simulink model "ntc_measure"  (R2024a)
settings: Solver=ode1be  StartTime=0.0  StopTime=simlength  FixedStep=tc  RelTol=1e-3
undefined symbols (not defined in the file or in its folder): open_loop_gain_opa350, Rntc, tc
libraries: fl_lib x177, ee_lib x28, nesl_utility x26
(part 1 of 2)
settings Model: SimulationMode=accelerator  Creator=ltnbda  LastModifiedBy=ltnbda
settings DataIOCC: SaveOutput=off  SignalLogging=off  DSMLogging=off  SaveTime=off  ReturnWorkspaceOutputs=off
settings RTWCC: GPUComputeCapability=3.5

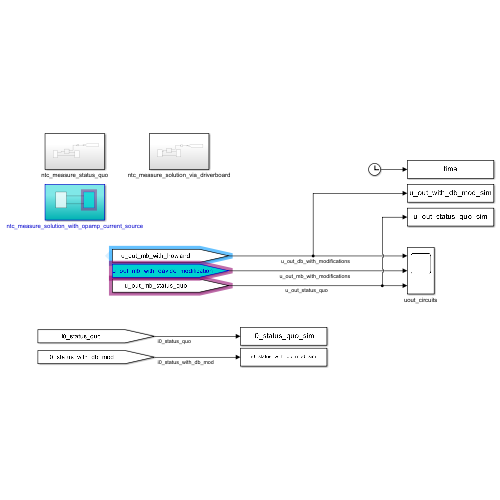
[thumbnail: Simulink's stored preview of the top-level diagram]
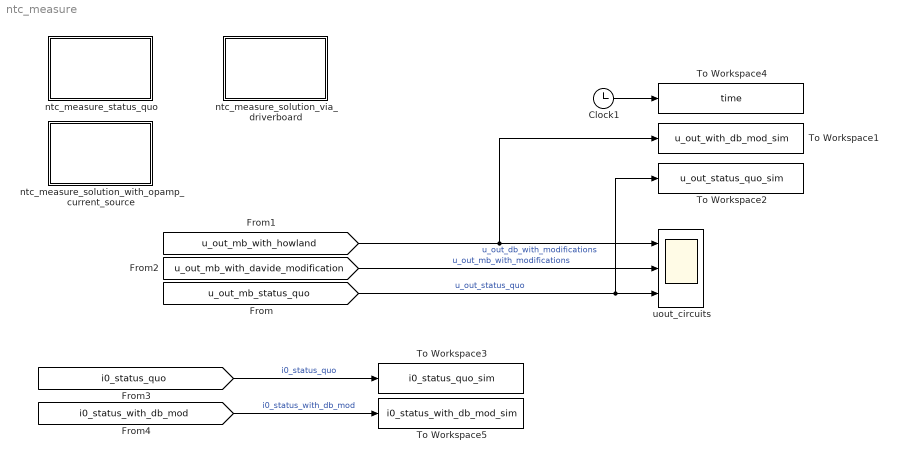
== system ntc_measure ==
  Clock1 : Clock
  To Workspace1 : ToWorkspace  VariableName=u_out_with_db_mod_sim  SampleTime=tc
      settings: MaxDataPoints=Nc
  To Workspace2 : ToWorkspace  VariableName=u_out_status_quo_sim  SampleTime=tc
      settings: MaxDataPoints=Nc
  To Workspace3 : ToWorkspace  VariableName=i0_status_quo_sim  SampleTime=tc
      settings: MaxDataPoints=Nc
  To Workspace4 : ToWorkspace  VariableName=time  SampleTime=tc
      settings: MaxDataPoints=Nc
  To Workspace5 : ToWorkspace  VariableName=i0_status_with_db_mod_sim  SampleTime=tc
      settings: MaxDataPoints=Nc
  ntc_measure_solution_via_driverboard : Subsystem
  ntc_measure_solution_with_opamp_current_source : Subsystem
  ntc_measure_status_quo : Subsystem
  uout_circuits : Scope  NumInputPorts=3
  wires:
  [u_out_mb_with_howland] -> To Workspace1/1, uout_circuits/1  "u_out_db_with_modifications"
  [u_out_mb_with_davide_modification] -> uout_circuits/2  "u_out_mb_with_modifications"
  [u_out_mb_status_quo] -> To Workspace2/1, uout_circuits/3  "u_out_status_quo"
  Clock1/1 -> To Workspace4/1
  [i0_status_quo] -> To Workspace3/1  "i0_status_quo"
  [i0_status_with_db_mod] -> To Workspace5/1  "i0_status_with_db_mod"

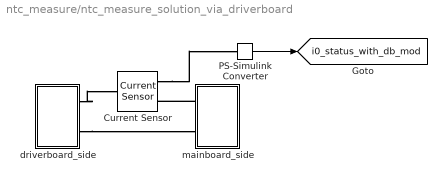
== system ntc_measure/ntc_measure_solution_via_driverboard ==
  Current Sensor : fl_lib/Electrical/Electrical Sensors/Current Sensor
  PS-Simulink Converter : nesl_utility/PS-Simulink Converter  PhysicalDomain=network_engine_domain  SubClassName=ps_output  LeftPortType=input  RightPortType=output  PseudoPeriodic=off  Frequencies=[]  VectorFormat=1-D array  Unit=A  AffineConversion=off
  driverboard_side : Subsystem
  mainboard_side : Subsystem
  tag scope: i0_status_with_db_mod=global
  wires:
  PS-Simulink Converter/1 -> [i0_status_with_db_mod]
  connections:
  driverboard_side/RConn2 -- mainboard_side/LConn2
  Current Sensor/RConn1 -- PS-Simulink Converter/LConn1
  mainboard_side/LConn1 -- Current Sensor/RConn2
  driverboard_side/RConn1 -- Current Sensor/LConn1

== system ntc_measure/ntc_measure_solution_with_opamp_current_source ==
  driverboard_side : Subsystem
  mainboard_side : Subsystem
  connections:
  mainboard_side/LConn2 -- driverboard_side/RConn2
  mainboard_side/LConn1 -- driverboard_side/RConn1

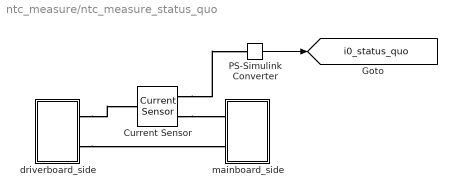
== system ntc_measure/ntc_measure_status_quo ==
  Current Sensor : fl_lib/Electrical/Electrical Sensors/Current Sensor
  PS-Simulink Converter : nesl_utility/PS-Simulink Converter  PhysicalDomain=network_engine_domain  SubClassName=ps_output  LeftPortType=input  RightPortType=output  PseudoPeriodic=off  Frequencies=[]  VectorFormat=1-D array  Unit=A  AffineConversion=off
  driverboard_side : Subsystem
  mainboard_side : Subsystem
  tag scope: i0_status_quo=global
  wires:
  PS-Simulink Converter/1 -> [i0_status_quo]
  connections:
  driverboard_side/RConn2 -- mainboard_side/LConn2
  driverboard_side/RConn1 -- Current Sensor/LConn1
  Current Sensor/RConn2 -- mainboard_side/LConn1
  Current Sensor/RConn1 -- PS-Simulink Converter/LConn1

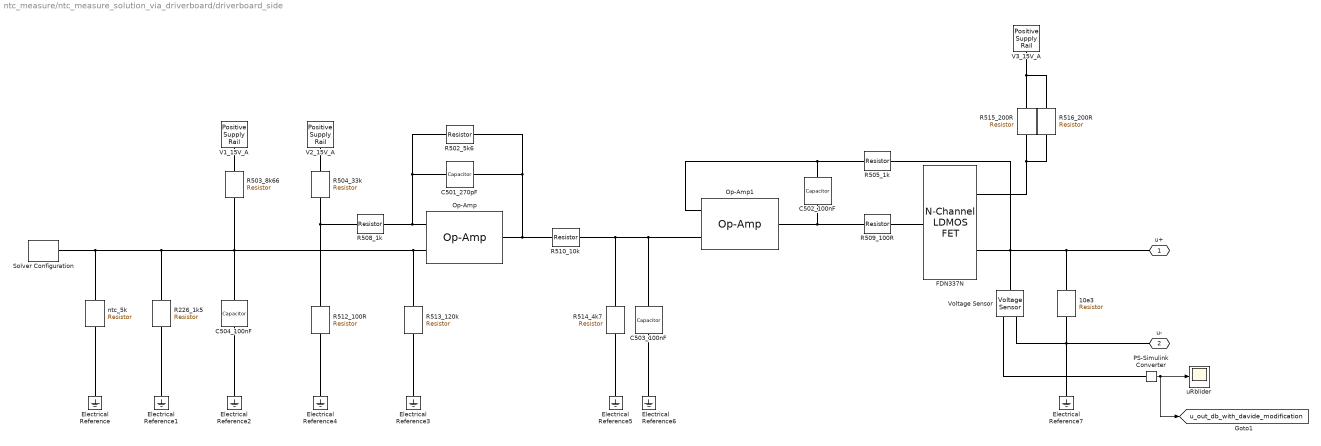
== system ntc_measure/ntc_measure_solution_via_driverboard/driverboard_side ==
  10e3 : fl_lib/Electrical/Electrical Elements/Resistor  R=10e3 Ohm  i_specify=off  i_priority=None  i=0 A  i_nominal_specify=off  i_nominal_value=1  i_nominal_unit=A  v_specify=off  v_priority=None  v=0 V  v_nominal_specify=off  v_nominal_value=1  v_nominal_unit=V
  C501_270pF : fl_lib/Electrical/Electrical Elements/Capacitor  c=270e-12 F  r=1e-6 Ohm  g=0 1/Ohm  i_specify=off  i_priority=None  i=0 A  i_nominal_specify=off  i_nominal_value=1  i_nominal_unit=A  v_specify=off  v_priority=None  v=0 V  v_nominal_specify=off  v_nominal_value=1  v_nominal_unit=V  vc_specify=off  vc_priority=High  vc=0 V  vc_nominal_specify=off  vc_nominal_value=1  vc_nominal_unit=V
  C502_100nF : fl_lib/Electrical/Electrical Elements/Capacitor  c=100e-9 F  r=1e-6 Ohm  g=0 1/Ohm  i_specify=off  i_priority=None  i=0 A  i_nominal_specify=off  i_nominal_value=1  i_nominal_unit=A  v_specify=off  v_priority=None  v=0 V  v_nominal_specify=off  v_nominal_value=1  v_nominal_unit=V  vc_specify=off  vc_priority=High  vc=0 V  vc_nominal_specify=off  vc_nominal_value=1  vc_nominal_unit=V
  C503_100nF : fl_lib/Electrical/Electrical Elements/Capacitor  c=100e-9 F  r=1e-6 Ohm  g=0 1/Ohm  i_specify=off  i_priority=None  i=0 A  i_nominal_specify=off  i_nominal_value=1  i_nominal_unit=A  v_specify=off  v_priority=None  v=0 V  v_nominal_specify=off  v_nominal_value=1  v_nominal_unit=V  vc_specify=off  vc_priority=High  vc=0 V  vc_nominal_specify=off  vc_nominal_value=1  vc_nominal_unit=V
  C504_100nF : fl_lib/Electrical/Electrical Elements/Capacitor  c=100e-9 F  r=1e-6 Ohm  g=0 1/Ohm  i_specify=off  i_priority=None  i=0 A  i_nominal_specify=off  i_nominal_value=1  i_nominal_unit=A  v_specify=off  v_priority=None  v=0 V  v_nominal_specify=off  v_nominal_value=1  v_nominal_unit=V  vc_specify=off  vc_priority=High  vc=0 V  vc_nominal_specify=off  vc_nominal_value=1  vc_nominal_unit=V
  Electrical Reference{,1..7} (8 alike) : fl_lib/Electrical/Electrical Elements/Electrical Reference
  FDN337N : ee_lib/Semiconductors & Converters/N-Channel LDMOS FET  betaref=[11.6, .01] A/V^2  Vfbref=[-1.05, -.1] V  gamma=[3.4, 2.5] V^(1/2)  phib2ref=[.95, .95] V  thesatref=[0, .1] 1/V  theaccdr=0 1/V  alpha=0  Vp=5e-2 V  m=8  Tmeas=25 degC  Rsref=1e-4 Ohm  Rdref=0.07 Ohm  Rgref=8.4 Ohm  Rdriftref=0.1 Ohm  lambda=0.2  Cox=[1600, 1000] pF  Cgso=15 pF  Cgdo=15 pF  Isref=1e-13 A  Vbi=0.6 V  n=1  Cj0=1800 pF  TT=50e-9 s  Tprm=1  Tsim=25 degC  etabet=[1.3, 1.3]  Stvfb=[.0005, .0005] V/K  Stphib=-8.5e-4 V/K  etasat=[1.04, 1.04]  etar=0.95  etardr=0.95  etais=3  Ig_specify=off  Ig_priority=None  Ig=0 A  Ig_nominal_specify=off  Ig_nominal_value=1  Ig_nominal_unit=A  Id_specify=off  Id_priority=None  Id=0 A  Id_nominal_specify=off  Id_nominal_value=1  Id_nominal_unit=A  V_gs_specify=off  V_gs_priority=None  V_gs=0 V  V_gs_nominal_specify=off  V_gs_nominal_value=1  V_gs_nominal_unit=V  V_ds_specify=off  V_ds_priority=None  V_ds=0 V  V_ds_nominal_specify=off  V_ds_nominal_value=1  V_ds_nominal_unit=V  QGoverCox_specify=off  QGoverCox_priority=Low  QGoverCox=0 V  QGoverCox_nominal_specify=off  QGoverCox_nominal_value=1  QGoverCox_nominal_unit=V  QDoverCox_specify=off  QDoverCox_priority=Low  QDoverCox=0 V  QDoverCox_nominal_specify=off  QDoverCox_nominal_value=1  QDoverCox_nominal_unit=V  thermal_network_parameterization=ee.enum.thermalNetworkTopology.junctionCase  Rth=[0, 10] K/W  Rth_Cauer=[1, 3, 10] K/W  Rth_Foster=[4, 6] K/W  thermal_mass_parameterization=ee.enum.thermalNetwork.timeconstant  thermal_mass=[0, 1] J/K  thermal_mass_Cauer=[.1, .3, 1] J/K  thermal_mass_Foster=[1.5, 3] J/K  thermal_time_constant=[0, 10] s  thermal_time_constant_Cauer=[1, 3, 10] s  thermal_time_constant_Foster=[6, 18] s  T0=[25, 25] degC  T0_Cauer=[25, 25, 25] degC  Tvec_initial_Foster=[25, 25, 25, 25] degC
      settings: InternalSimscapePortConfiguration="{\"Bottom\":[],\"Left\":[{\"id\":\"G\",\"label\":\"\",\"type\":\"foundation.electrical.electrical\"}],\"Right\":[{\"id\":\"D\",\"label\":\"d\",\"type\":\"foundation.electrical.electrical\"},{\"id\":\"S\",\"label\":\"s\",\"type\":\"foundation.electrical.electrical\"}],\"Top\":[]}"
  Op-Amp : fl_lib/Electrical/Electrical Elements/Op-Amp  outI_specify=off  outI_priority=None  outI=0 A  outI_nominal_specify=off  outI_nominal_value=1  outI_nominal_unit=A
  Op-Amp1 : fl_lib/Electrical/Electrical Elements/Op-Amp  outI_specify=off  outI_priority=None  outI=0 A  outI_nominal_specify=off  outI_nominal_value=1  outI_nominal_unit=A
  PS-Simulink Converter : nesl_utility/PS-Simulink Converter  PhysicalDomain=network_engine_domain  SubClassName=ps_output  LeftPortType=input  RightPortType=output  PseudoPeriodic=off  Frequencies=[]  VectorFormat=1-D array  Unit=V  AffineConversion=off
  R226_1k5 : fl_lib/Electrical/Electrical Elements/Resistor  R=1.5e3 Ohm  i_specify=off  i_priority=None  i=0 A  i_nominal_specify=off  i_nominal_value=1  i_nominal_unit=A  v_specify=off  v_priority=None  v=0 V  v_nominal_specify=off  v_nominal_value=1  v_nominal_unit=V
  R502_5k6 : fl_lib/Electrical/Electrical Elements/Resistor  R=5.6e3 Ohm  i_specify=off  i_priority=None  i=0 A  i_nominal_specify=off  i_nominal_value=1  i_nominal_unit=A  v_specify=off  v_priority=None  v=0 V  v_nominal_specify=off  v_nominal_value=1  v_nominal_unit=V
  R503_8k66 : fl_lib/Electrical/Electrical Elements/Resistor  R=8.66e3 Ohm  i_specify=off  i_priority=None  i=0 A  i_nominal_specify=off  i_nominal_value=1  i_nominal_unit=A  v_specify=off  v_priority=None  v=0 V  v_nominal_specify=off  v_nominal_value=1  v_nominal_unit=V
  R504_33k : fl_lib/Electrical/Electrical Elements/Resistor  R=33e3 Ohm  i_specify=off  i_priority=None  i=0 A  i_nominal_specify=off  i_nominal_value=1  i_nominal_unit=A  v_specify=off  v_priority=None  v=0 V  v_nominal_specify=off  v_nominal_value=1  v_nominal_unit=V
  R505_1k : fl_lib/Electrical/Electrical Elements/Resistor  R=1e3 Ohm  i_specify=off  i_priority=None  i=0 A  i_nominal_specify=off  i_nominal_value=1  i_nominal_unit=A  v_specify=off  v_priority=None  v=0 V  v_nominal_specify=off  v_nominal_value=1  v_nominal_unit=V
  R508_1k : fl_lib/Electrical/Electrical Elements/Resistor  R=1e3 Ohm  i_specify=off  i_priority=None  i=0 A  i_nominal_specify=off  i_nominal_value=1  i_nominal_unit=A  v_specify=off  v_priority=None  v=0 V  v_nominal_specify=off  v_nominal_value=1  v_nominal_unit=V
  R509_100R : fl_lib/Electrical/Electrical Elements/Resistor  R=100 Ohm  i_specify=off  i_priority=None  i=0 A  i_nominal_specify=off  i_nominal_value=1  i_nominal_unit=A  v_specify=off  v_priority=None  v=0 V  v_nominal_specify=off  v_nominal_value=1  v_nominal_unit=V
  R510_10k : fl_lib/Electrical/Electrical Elements/Resistor  R=10e3 Ohm  i_specify=off  i_priority=None  i=0 A  i_nominal_specify=off  i_nominal_value=1  i_nominal_unit=A  v_specify=off  v_priority=None  v=0 V  v_nominal_specify=off  v_nominal_value=1  v_nominal_unit=V
  R512_100R : fl_lib/Electrical/Electrical Elements/Resistor  R=100 Ohm  i_specify=off  i_priority=None  i=0 A  i_nominal_specify=off  i_nominal_value=1  i_nominal_unit=A  v_specify=off  v_priority=None  v=0 V  v_nominal_specify=off  v_nominal_value=1  v_nominal_unit=V
  R513_120k : fl_lib/Electrical/Electrical Elements/Resistor  R=120e3 Ohm  i_specify=off  i_priority=None  i=0 A  i_nominal_specify=off  i_nominal_value=1  i_nominal_unit=A  v_specify=off  v_priority=None  v=0 V  v_nominal_specify=off  v_nominal_value=1  v_nominal_unit=V
  R514_4k7 : fl_lib/Electrical/Electrical Elements/Resistor  R=4.7e3 Ohm  i_specify=off  i_priority=None  i=0 A  i_nominal_specify=off  i_nominal_value=1  i_nominal_unit=A  v_specify=off  v_priority=None  v=0 V  v_nominal_specify=off  v_nominal_value=1  v_nominal_unit=V
  R515_200R : fl_lib/Electrical/Electrical Elements/Resistor  R=200 Ohm  i_specify=off  i_priority=None  i=0 A  i_nominal_specify=off  i_nominal_value=1  i_nominal_unit=A  v_specify=off  v_priority=None  v=0 V  v_nominal_specify=off  v_nominal_value=1  v_nominal_unit=V
  R516_200R : fl_lib/Electrical/Electrical Elements/Resistor  R=200 Ohm  i_specify=off  i_priority=None  i=0 A  i_nominal_specify=off  i_nominal_value=1  i_nominal_unit=A  v_specify=off  v_priority=None  v=0 V  v_nominal_specify=off  v_nominal_value=1  v_nominal_unit=V
  Solver Configuration : nesl_utility/Solver Configuration  PhysicalDomain=network_engine_domain  SubClassName=solver  LeftPortType=input  RightPortType=generic  Tones=[]  Harmonics=[]  SimulateNoise=off  Profile=off  UseLocalSampling=off  EnableSwitchedLinearOptims=on  FrequencyDomain=off  UseCCode=off  RelTol=0.001  AbsTol=0.001  MinStep=1e-09  ToWorkspace=off  RevertToSquareIcSolve=off  NumHomotopyIterations=100  PhasorMode=off  PhasorModeNumHarmonics=1  ConsistencySolver=NEWTON_XTOL_AFTER_FTOL  IndexReductionMethod=DerivativeReplacement  DoDC=off  ResidualTolerance=1e-09  ConsistencyTolSource=GLOBAL  ConsistencyAbsTol=0.001  ConsistencyRelTol=0.001  ConsistencyTolFactor=0.001  UseLocalSolver=on  LocalSolverChoice=NE_BACKWARD_EULER_ADVANCER  ResolveIndetEquations=on  FunctionEvalNumThread=1  LocalSolverSampleTime=tc  DoFixedCost=on  MaxNonlinIter=3  MaxModeIter=2  ComputeImpulses=off  ImpulseIterations=2  LinearAlgebra=auto  LinearAlgebraNumThread=0  EquationFormulation=NE_TIME_EF  DelaysMemoryBudget=1024  AutomaticFiltering=on  FilteringTimeConstant=0.001  PartitionStorageMethod=AS_NEEDED  PartitionMemoryBudget=1024  PartitionMethod=ROBUST  MultibodyUseLocalSolver=off  MultibodyLocalSolverChoice=ODE1  MultibodyLocalSolverSampleTime=0.001
  V1_15V_A : ee_lib/Sources/Positive Supply Rail  v0=15 V
      settings: InternalSimscapePortConfiguration="{\"Bottom\":[],\"Left\":[],\"Right\":[{\"id\":\"p\",\"label\":\"\",\"type\":\"foundation.electrical.electrical\"}],\"Top\":[]}"
  V2_15V_A : ee_lib/Sources/Positive Supply Rail  v0=15 V
      settings: InternalSimscapePortConfiguration="{\"Bottom\":[],\"Left\":[],\"Right\":[{\"id\":\"p\",\"label\":\"\",\"type\":\"foundation.electrical.electrical\"}],\"Top\":[]}"
  V3_15V_A : ee_lib/Sources/Positive Supply Rail  v0=15 V
      settings: InternalSimscapePortConfiguration="{\"Bottom\":[],\"Left\":[],\"Right\":[{\"id\":\"p\",\"label\":\"\",\"type\":\"foundation.electrical.electrical\"}],\"Top\":[]}"
  Voltage Sensor : fl_lib/Electrical/Electrical Sensors/Voltage Sensor
  ntc_5k : fl_lib/Electrical/Electrical Elements/Resistor  R=Rntc Ohm  i_specify=off  i_priority=None  i=0 A  i_nominal_specify=off  i_nominal_value=1  i_nominal_unit=A  v_specify=off  v_priority=None  v=0 V  v_nominal_specify=off  v_nominal_value=1  v_nominal_unit=V
  uRblider : Scope
  u+ : PMIOPort  Side=Right
  u- : PMIOPort  Port=2  Side=Right
  tag scope: u_out_db_with_davide_modification=global
  wires:
  PS-Simulink Converter/1 -> [u_out_db_with_davide_modification], uRblider/1
  connections:
  PS-Simulink Converter/LConn1 -- Voltage Sensor/RConn1
  Electrical Reference4/LConn1 -- R512_100R/RConn1
  Electrical Reference3/LConn1 -- R513_120k/RConn1
  Electrical Reference6/LConn1 -- C503_100nF/RConn1
  R502_5k6/RConn1 -- Op-Amp/RConn1 -- R510_10k/LConn1 -- C501_270pF/RConn1
  R514_4k7/LConn1 -- Op-Amp1/LConn1 -- C503_100nF/LConn1 -- R510_10k/RConn1
  Electrical Reference2/LConn1 -- C504_100nF/RConn1
  Electrical Reference1/LConn1 -- R226_1k5/RConn1
  V1_15V_A/RConn1 -- R503_8k66/LConn1
  Electrical Reference/LConn1 -- ntc_5k/RConn1
  R509_100R/LConn1 -- C502_100nF/RConn1 -- Op-Amp1/RConn1
  u+/RConn1 -- 10e3/LConn1 -- FDN337N/RConn2 -- Voltage Sensor/LConn1 -- R505_1k/RConn1
  FDN337N/LConn1 -- R509_100R/RConn1
  C501_270pF/LConn1 -- R502_5k6/LConn1 -- Op-Amp/LConn2 -- R508_1k/RConn1
  R505_1k/LConn1 -- C502_100nF/LConn1 -- Op-Amp1/LConn2
  R504_33k/LConn1 -- V2_15V_A/RConn1
  Voltage Sensor/RConn2 -- Electrical Reference7/LConn1 -- 10e3/RConn1 -- u-/RConn1
  Electrical Reference5/LConn1 -- R514_4k7/RConn1
  C504_100nF/LConn1 -- R513_120k/LConn1 -- Op-Amp/LConn1 -- Solver Configuration/RConn1 -- ntc_5k/LConn1 -- R226_1k5/LConn1 -- R503_8k66/RConn1
  R504_33k/RConn1 -- R512_100R/LConn1 -- R508_1k/LConn1
  R515_200R/LConn1 -- R516_200R/LConn1 -- V3_15V_A/RConn1
  FDN337N/RConn1 -- R516_200R/RConn1 -- R515_200R/RConn1

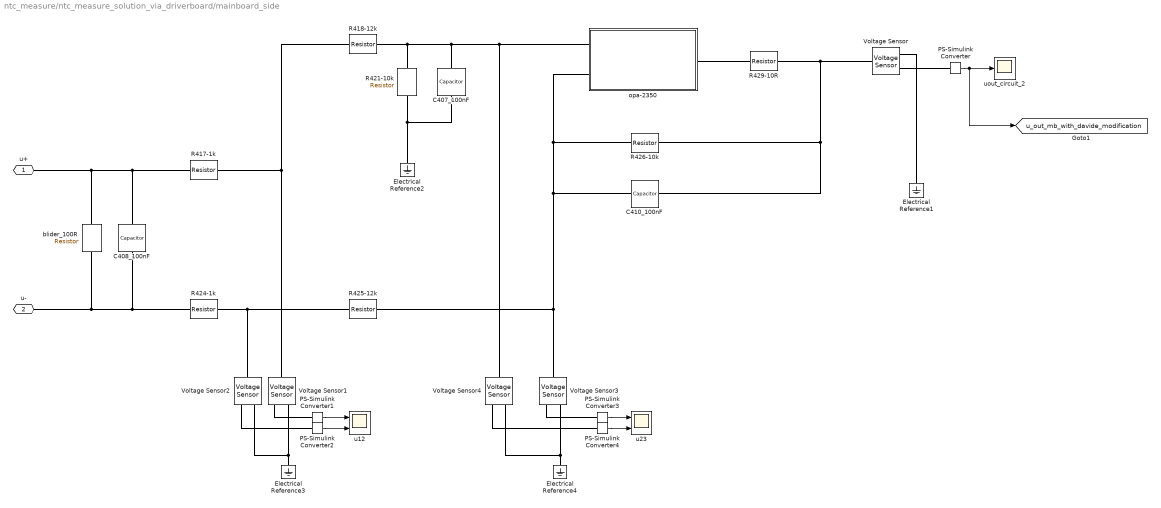
== system ntc_measure/ntc_measure_solution_via_driverboard/mainboard_side ==
  C407_100nF : fl_lib/Electrical/Electrical Elements/Capacitor  c=100e-9 F  r=1e-6 Ohm  g=0 1/Ohm  i_specify=off  i_priority=None  i=0 A  i_nominal_specify=off  i_nominal_value=1  i_nominal_unit=A  v_specify=off  v_priority=None  v=0 V  v_nominal_specify=off  v_nominal_value=1  v_nominal_unit=V  vc_specify=off  vc_priority=High  vc=0 V  vc_nominal_specify=off  vc_nominal_value=1  vc_nominal_unit=V
  C408_100nF : fl_lib/Electrical/Electrical Elements/Capacitor  c=100e-9 F  r=1e-6 Ohm  g=0 1/Ohm  i_specify=off  i_priority=None  i=0 A  i_nominal_specify=off  i_nominal_value=1  i_nominal_unit=A  v_specify=off  v_priority=None  v=0 V  v_nominal_specify=off  v_nominal_value=1  v_nominal_unit=V  vc_specify=off  vc_priority=High  vc=0 V  vc_nominal_specify=off  vc_nominal_value=1  vc_nominal_unit=V
  C410_100nF : fl_lib/Electrical/Electrical Elements/Capacitor  c=100e-9 F  r=1e-6 Ohm  g=0 1/Ohm  i_specify=off  i_priority=None  i=0 A  i_nominal_specify=off  i_nominal_value=1  i_nominal_unit=A  v_specify=off  v_priority=None  v=0 V  v_nominal_specify=off  v_nominal_value=1  v_nominal_unit=V  vc_specify=off  vc_priority=High  vc=0 V  vc_nominal_specify=off  vc_nominal_value=1  vc_nominal_unit=V
  Electrical Reference{1..4} (4 alike) : fl_lib/Electrical/Electrical Elements/Electrical Reference
  PS-Simulink Converter{,1..4} (5 alike) : nesl_utility/PS-Simulink Converter  PhysicalDomain=network_engine_domain  SubClassName=ps_output  LeftPortType=input  RightPortType=output  PseudoPeriodic=off  Frequencies=[]  VectorFormat=1-D array  Unit=V  AffineConversion=off
  R417-1k : fl_lib/Electrical/Electrical Elements/Resistor  R=1e3 Ohm  i_specify=off  i_priority=None  i=0 A  i_nominal_specify=off  i_nominal_value=1  i_nominal_unit=A  v_specify=off  v_priority=None  v=0 V  v_nominal_specify=off  v_nominal_value=1  v_nominal_unit=V
  R418-12k : fl_lib/Electrical/Electrical Elements/Resistor  R=12e3 Ohm  i_specify=off  i_priority=None  i=0 A  i_nominal_specify=off  i_nominal_value=1  i_nominal_unit=A  v_specify=off  v_priority=None  v=0 V  v_nominal_specify=off  v_nominal_value=1  v_nominal_unit=V
  R421-10k : fl_lib/Electrical/Electrical Elements/Resistor  R=10e3 Ohm  i_specify=off  i_priority=None  i=0 A  i_nominal_specify=off  i_nominal_value=1  i_nominal_unit=A  v_specify=off  v_priority=None  v=0 V  v_nominal_specify=off  v_nominal_value=1  v_nominal_unit=V
  R424-1k : fl_lib/Electrical/Electrical Elements/Resistor  R=1e3 Ohm  i_specify=off  i_priority=None  i=0 A  i_nominal_specify=off  i_nominal_value=1  i_nominal_unit=A  v_specify=off  v_priority=None  v=0 V  v_nominal_specify=off  v_nominal_value=1  v_nominal_unit=V
  R425-12k : fl_lib/Electrical/Electrical Elements/Resistor  R=12e3 Ohm  i_specify=off  i_priority=None  i=0 A  i_nominal_specify=off  i_nominal_value=1  i_nominal_unit=A  v_specify=off  v_priority=None  v=0 V  v_nominal_specify=off  v_nominal_value=1  v_nominal_unit=V
  R426-10k : fl_lib/Electrical/Electrical Elements/Resistor  R=10e3 Ohm  i_specify=off  i_priority=None  i=0 A  i_nominal_specify=off  i_nominal_value=1  i_nominal_unit=A  v_specify=off  v_priority=None  v=0 V  v_nominal_specify=off  v_nominal_value=1  v_nominal_unit=V
  R429-10R : fl_lib/Electrical/Electrical Elements/Resistor  R=10 Ohm  i_specify=off  i_priority=None  i=0 A  i_nominal_specify=off  i_nominal_value=1  i_nominal_unit=A  v_specify=off  v_priority=None  v=0 V  v_nominal_specify=off  v_nominal_value=1  v_nominal_unit=V
  Voltage Sensor{,1..4} (5 alike) : fl_lib/Electrical/Electrical Sensors/Voltage Sensor
  blider_100R : fl_lib/Electrical/Electrical Elements/Resistor  R=100 Ohm  i_specify=off  i_priority=None  i=0 A  i_nominal_specify=off  i_nominal_value=1  i_nominal_unit=A  v_specify=off  v_priority=None  v=0 V  v_nominal_specify=off  v_nominal_value=1  v_nominal_unit=V
  opa-2350 : Subsystem  mask{V_opamp_pos=3.6, V_opamp_neg=-1.6, A=1e6 %open_loop_gain_opa350}
      mask prompts: V_opamp_pos "V+"; V_opamp_neg "V-"; A "Open Loop Gain"
      mask help: rail to rail op-amp
      mask Help: eval('open opa2350.pdf')
      mask Display:
      | disp('OPA-2350');
      | port_label('lconn', 1, 'in(+)');
      | port_label('lconn', 2, 'in(-)');
      | port_label('rconn', 1, 'out');
  u12 : Scope  NumInputPorts=2
  u23 : Scope  NumInputPorts=2
  uout_circuit_2 : Scope
  u+ : PMIOPort  Side=Left
  u- : PMIOPort  Port=2  Side=Left
  tag scope: u_out_mb_with_davide_modification=global
  wires:
  PS-Simulink Converter3/1 -> u23/1
  PS-Simulink Converter4/1 -> u23/2
  PS-Simulink Converter2/1 -> u12/2
  PS-Simulink Converter1/1 -> u12/1
  PS-Simulink Converter/1 -> [u_out_mb_with_davide_modification], uout_circuit_2/1
  connections:
  Voltage Sensor3/RConn1 -- PS-Simulink Converter3/LConn1
  Voltage Sensor4/RConn1 -- PS-Simulink Converter4/LConn1
  Voltage Sensor4/RConn2 -- Electrical Reference4/LConn1 -- Voltage Sensor3/RConn2
  Voltage Sensor2/RConn1 -- PS-Simulink Converter2/LConn1
  Electrical Reference3/LConn1 -- Voltage Sensor2/RConn2 -- Voltage Sensor1/RConn2
  Voltage Sensor1/RConn1 -- PS-Simulink Converter1/LConn1
  PS-Simulink Converter/LConn1 -- Voltage Sensor/RConn1
  Voltage Sensor/RConn2 -- Electrical Reference1/LConn1
  Voltage Sensor/LConn1 -- R426-10k/RConn1 -- C410_100nF/RConn1 -- R429-10R/RConn1
  R421-10k/RConn1 -- C407_100nF/RConn1 -- Electrical Reference2/LConn1
  R418-12k/LConn1 -- R421-10k/LConn1 -- C407_100nF/LConn1 -- Voltage Sensor4/LConn1 -- opa-2350/LConn1
  R425-12k/RConn1 -- R424-1k/LConn1 -- Voltage Sensor2/LConn1
  R418-12k/RConn1 -- R417-1k/LConn1 -- Voltage Sensor1/LConn1
  C408_100nF/RConn1 -- R424-1k/RConn1 -- blider_100R/RConn1 -- u-/RConn1
  C408_100nF/LConn1 -- R417-1k/RConn1 -- blider_100R/LConn1 -- u+/RConn1
  R426-10k/LConn1 -- Voltage Sensor3/LConn1 -- R425-12k/LConn1 -- C410_100nF/LConn1 -- opa-2350/LConn2
  R429-10R/LConn1 -- opa-2350/RConn1

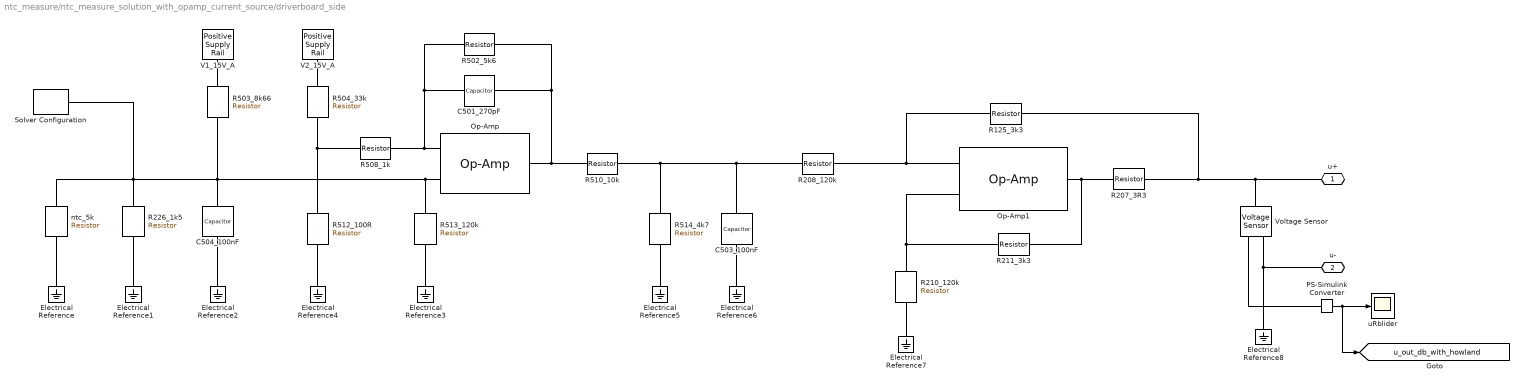
== system ntc_measure/ntc_measure_solution_with_opamp_current_source/driverboard_side ==
  C501_270pF : fl_lib/Electrical/Electrical Elements/Capacitor  c=270e-12 F  r=1e-6 Ohm  g=0 1/Ohm  i_specify=off  i_priority=None  i=0 A  i_nominal_specify=off  i_nominal_value=1  i_nominal_unit=A  v_specify=off  v_priority=None  v=0 V  v_nominal_specify=off  v_nominal_value=1  v_nominal_unit=V  vc_specify=off  vc_priority=High  vc=0 V  vc_nominal_specify=off  vc_nominal_value=1  vc_nominal_unit=V
  C503_100nF : fl_lib/Electrical/Electrical Elements/Capacitor  c=100e-9 F  r=1e-6 Ohm  g=0 1/Ohm  i_specify=off  i_priority=None  i=0 A  i_nominal_specify=off  i_nominal_value=1  i_nominal_unit=A  v_specify=off  v_priority=None  v=0 V  v_nominal_specify=off  v_nominal_value=1  v_nominal_unit=V  vc_specify=off  vc_priority=High  vc=0 V  vc_nominal_specify=off  vc_nominal_value=1  vc_nominal_unit=V
  C504_100nF : fl_lib/Electrical/Electrical Elements/Capacitor  c=100e-9 F  r=1e-6 Ohm  g=0 1/Ohm  i_specify=off  i_priority=None  i=0 A  i_nominal_specify=off  i_nominal_value=1  i_nominal_unit=A  v_specify=off  v_priority=None  v=0 V  v_nominal_specify=off  v_nominal_value=1  v_nominal_unit=V  vc_specify=off  vc_priority=High  vc=0 V  vc_nominal_specify=off  vc_nominal_value=1  vc_nominal_unit=V
  Electrical Reference{,1..8} (9 alike) : fl_lib/Electrical/Electrical Elements/Electrical Reference
  Op-Amp : fl_lib/Electrical/Electrical Elements/Op-Amp  outI_specify=off  outI_priority=None  outI=0 A  outI_nominal_specify=off  outI_nominal_value=1  outI_nominal_unit=A
  Op-Amp1 : fl_lib/Electrical/Electrical Elements/Op-Amp  outI_specify=off  outI_priority=None  outI=0 A  outI_nominal_specify=off  outI_nominal_value=1  outI_nominal_unit=A
  PS-Simulink Converter : nesl_utility/PS-Simulink Converter  PhysicalDomain=network_engine_domain  SubClassName=ps_output  LeftPortType=input  RightPortType=output  PseudoPeriodic=off  Frequencies=[]  VectorFormat=1-D array  Unit=V  AffineConversion=off
  R125_3k3 : fl_lib/Electrical/Electrical Elements/Resistor  R=3.3e3 Ohm  i_specify=off  i_priority=None  i=0 A  i_nominal_specify=off  i_nominal_value=1  i_nominal_unit=A  v_specify=off  v_priority=None  v=0 V  v_nominal_specify=off  v_nominal_value=1  v_nominal_unit=V
  R207_3R3 : fl_lib/Electrical/Electrical Elements/Resistor  R=3.3 Ohm  i_specify=off  i_priority=None  i=0 A  i_nominal_specify=off  i_nominal_value=1  i_nominal_unit=A  v_specify=off  v_priority=None  v=0 V  v_nominal_specify=off  v_nominal_value=1  v_nominal_unit=V
  R208_120k : fl_lib/Electrical/Electrical Elements/Resistor  R=120e3 Ohm  i_specify=off  i_priority=None  i=0 A  i_nominal_specify=off  i_nominal_value=1  i_nominal_unit=A  v_specify=off  v_priority=None  v=0 V  v_nominal_specify=off  v_nominal_value=1  v_nominal_unit=V
  R210_120k : fl_lib/Electrical/Electrical Elements/Resistor  R=120e3 Ohm  i_specify=off  i_priority=None  i=0 A  i_nominal_specify=off  i_nominal_value=1  i_nominal_unit=A  v_specify=off  v_priority=None  v=0 V  v_nominal_specify=off  v_nominal_value=1  v_nominal_unit=V
  R211_3k3 : fl_lib/Electrical/Electrical Elements/Resistor  R=3.3e3 Ohm  i_specify=off  i_priority=None  i=0 A  i_nominal_specify=off  i_nominal_value=1  i_nominal_unit=A  v_specify=off  v_priority=None  v=0 V  v_nominal_specify=off  v_nominal_value=1  v_nominal_unit=V
  R226_1k5 : fl_lib/Electrical/Electrical Elements/Resistor  R=1.5e3 Ohm  i_specify=off  i_priority=None  i=0 A  i_nominal_specify=off  i_nominal_value=1  i_nominal_unit=A  v_specify=off  v_priority=None  v=0 V  v_nominal_specify=off  v_nominal_value=1  v_nominal_unit=V
  R502_5k6 : fl_lib/Electrical/Electrical Elements/Resistor  R=5.6e3 Ohm  i_specify=off  i_priority=None  i=0 A  i_nominal_specify=off  i_nominal_value=1  i_nominal_unit=A  v_specify=off  v_priority=None  v=0 V  v_nominal_specify=off  v_nominal_value=1  v_nominal_unit=V
  R503_8k66 : fl_lib/Electrical/Electrical Elements/Resistor  R=8.66e3 Ohm  i_specify=off  i_priority=None  i=0 A  i_nominal_specify=off  i_nominal_value=1  i_nominal_unit=A  v_specify=off  v_priority=None  v=0 V  v_nominal_specify=off  v_nominal_value=1  v_nominal_unit=V
  R504_33k : fl_lib/Electrical/Electrical Elements/Resistor  R=33e3 Ohm  i_specify=off  i_priority=None  i=0 A  i_nominal_specify=off  i_nominal_value=1  i_nominal_unit=A  v_specify=off  v_priority=None  v=0 V  v_nominal_specify=off  v_nominal_value=1  v_nominal_unit=V
  R508_1k : fl_lib/Electrical/Electrical Elements/Resistor  R=1e3 Ohm  i_specify=off  i_priority=None  i=0 A  i_nominal_specify=off  i_nominal_value=1  i_nominal_unit=A  v_specify=off  v_priority=None  v=0 V  v_nominal_specify=off  v_nominal_value=1  v_nominal_unit=V
  R510_10k : fl_lib/Electrical/Electrical Elements/Resistor  R=10e3 Ohm  i_specify=off  i_priority=None  i=0 A  i_nominal_specify=off  i_nominal_value=1  i_nominal_unit=A  v_specify=off  v_priority=None  v=0 V  v_nominal_specify=off  v_nominal_value=1  v_nominal_unit=V
  R512_100R : fl_lib/Electrical/Electrical Elements/Resistor  R=100 Ohm  i_specify=off  i_priority=None  i=0 A  i_nominal_specify=off  i_nominal_value=1  i_nominal_unit=A  v_specify=off  v_priority=None  v=0 V  v_nominal_specify=off  v_nominal_value=1  v_nominal_unit=V
  R513_120k : fl_lib/Electrical/Electrical Elements/Resistor  R=120e3 Ohm  i_specify=off  i_priority=None  i=0 A  i_nominal_specify=off  i_nominal_value=1  i_nominal_unit=A  v_specify=off  v_priority=None  v=0 V  v_nominal_specify=off  v_nominal_value=1  v_nominal_unit=V
  R514_4k7 : fl_lib/Electrical/Electrical Elements/Resistor  R=4.7e3 Ohm  i_specify=off  i_priority=None  i=0 A  i_nominal_specify=off  i_nominal_value=1  i_nominal_unit=A  v_specify=off  v_priority=None  v=0 V  v_nominal_specify=off  v_nominal_value=1  v_nominal_unit=V
  Solver Configuration : nesl_utility/Solver Configuration  PhysicalDomain=network_engine_domain  SubClassName=solver  LeftPortType=input  RightPortType=generic  Tones=[]  Harmonics=[]  SimulateNoise=off  Profile=off  UseLocalSampling=off  EnableSwitchedLinearOptims=on  FrequencyDomain=off  UseCCode=off  RelTol=0.001  AbsTol=0.001  MinStep=1e-09  ToWorkspace=off  RevertToSquareIcSolve=off  NumHomotopyIterations=100  PhasorMode=off  PhasorModeNumHarmonics=1  ConsistencySolver=NEWTON_XTOL_AFTER_FTOL  IndexReductionMethod=DerivativeReplacement  DoDC=off  ResidualTolerance=1e-09  ConsistencyTolSource=GLOBAL  ConsistencyAbsTol=0.001  ConsistencyRelTol=0.001  ConsistencyTolFactor=0.001  UseLocalSolver=on  LocalSolverChoice=NE_BACKWARD_EULER_ADVANCER  ResolveIndetEquations=on  FunctionEvalNumThread=1  LocalSolverSampleTime=tc  DoFixedCost=on  MaxNonlinIter=3  MaxModeIter=2  ComputeImpulses=off  ImpulseIterations=2  LinearAlgebra=auto  LinearAlgebraNumThread=0  EquationFormulation=NE_TIME_EF  DelaysMemoryBudget=1024  AutomaticFiltering=on  FilteringTimeConstant=0.001  PartitionStorageMethod=AS_NEEDED  PartitionMemoryBudget=1024  PartitionMethod=ROBUST  MultibodyUseLocalSolver=off  MultibodyLocalSolverChoice=ODE1  MultibodyLocalSolverSampleTime=0.001
  V1_15V_A : ee_lib/Sources/Positive Supply Rail  v0=15 V
      settings: InternalSimscapePortConfiguration="{\"Bottom\":[],\"Left\":[],\"Right\":[{\"id\":\"p\",\"label\":\"\",\"type\":\"foundation.electrical.electrical\"}],\"Top\":[]}"
  V2_15V_A : ee_lib/Sources/Positive Supply Rail  v0=15 V
      settings: InternalSimscapePortConfiguration="{\"Bottom\":[],\"Left\":[],\"Right\":[{\"id\":\"p\",\"label\":\"\",\"type\":\"foundation.electrical.electrical\"}],\"Top\":[]}"
  Voltage Sensor : fl_lib/Electrical/Electrical Sensors/Voltage Sensor
  ntc_5k : fl_lib/Electrical/Electrical Elements/Resistor  R=Rntc Ohm  i_specify=off  i_priority=None  i=0 A  i_nominal_specify=off  i_nominal_value=1  i_nominal_unit=A  v_specify=off  v_priority=None  v=0 V  v_nominal_specify=off  v_nominal_value=1  v_nominal_unit=V
  uRblider : Scope
  u+ : PMIOPort  Side=Right
  u- : PMIOPort  Port=2  Side=Right
  tag scope: u_out_db_with_howland=global
  wires:
  PS-Simulink Converter/1 -> [u_out_db_with_howland], uRblider/1
  connections:
  PS-Simulink Converter/LConn1 -- Voltage Sensor/RConn1
  Electrical Reference4/LConn1 -- R512_100R/RConn1
  Electrical Reference3/LConn1 -- R513_120k/RConn1
  Electrical Reference6/LConn1 -- C503_100nF/RConn1
  R502_5k6/RConn1 -- Op-Amp/RConn1 -- R510_10k/LConn1 -- C501_270pF/RConn1
  R514_4k7/LConn1 -- C503_100nF/LConn1 -- R208_120k/LConn1 -- R510_10k/RConn1
  Electrical Reference2/LConn1 -- C504_100nF/RConn1
  Electrical Reference1/LConn1 -- R226_1k5/RConn1
  V1_15V_A/RConn1 -- R503_8k66/LConn1
  Electrical Reference/LConn1 -- ntc_5k/RConn1
  C501_270pF/LConn1 -- R502_5k6/LConn1 -- Op-Amp/LConn2 -- R508_1k/RConn1
  R504_33k/LConn1 -- V2_15V_A/RConn1
  Electrical Reference8/LConn1 -- u-/RConn1 -- Voltage Sensor/RConn2
  Electrical Reference5/LConn1 -- R514_4k7/RConn1
  C504_100nF/LConn1 -- R513_120k/LConn1 -- Op-Amp/LConn1 -- Solver Configuration/RConn1 -- ntc_5k/LConn1 -- R226_1k5/LConn1 -- R503_8k66/RConn1
  R504_33k/RConn1 -- R512_100R/LConn1 -- R508_1k/LConn1
  R125_3k3/RConn1 -- R207_3R3/RConn1 -- Voltage Sensor/LConn1 -- u+/RConn1
  R207_3R3/LConn1 -- R211_3k3/RConn1 -- Op-Amp1/RConn1
  R211_3k3/LConn1 -- Op-Amp1/LConn2 -- R210_120k/LConn1
  R125_3k3/LConn1 -- R208_120k/RConn1 -- Op-Amp1/LConn1
  Electrical Reference7/LConn1 -- R210_120k/RConn1

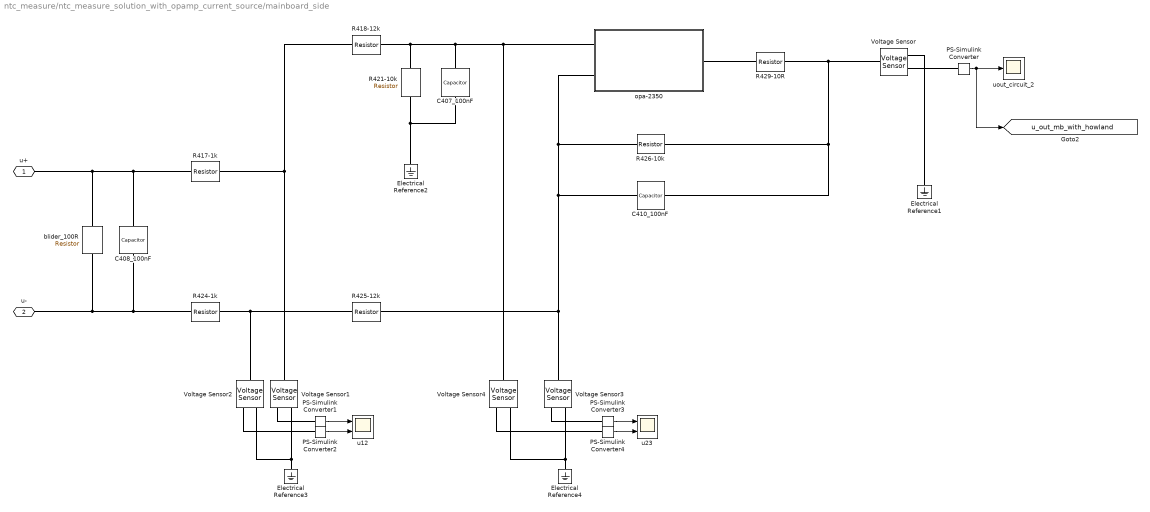
== system ntc_measure/ntc_measure_solution_with_opamp_current_source/mainboard_side ==
  C407_100nF : fl_lib/Electrical/Electrical Elements/Capacitor  c=100e-9 F  r=1e-6 Ohm  g=0 1/Ohm  i_specify=off  i_priority=None  i=0 A  i_nominal_specify=off  i_nominal_value=1  i_nominal_unit=A  v_specify=off  v_priority=None  v=0 V  v_nominal_specify=off  v_nominal_value=1  v_nominal_unit=V  vc_specify=off  vc_priority=High  vc=0 V  vc_nominal_specify=off  vc_nominal_value=1  vc_nominal_unit=V
  C408_100nF : fl_lib/Electrical/Electrical Elements/Capacitor  c=100e-9 F  r=1e-6 Ohm  g=0 1/Ohm  i_specify=off  i_priority=None  i=0 A  i_nominal_specify=off  i_nominal_value=1  i_nominal_unit=A  v_specify=off  v_priority=None  v=0 V  v_nominal_specify=off  v_nominal_value=1  v_nominal_unit=V  vc_specify=off  vc_priority=High  vc=0 V  vc_nominal_specify=off  vc_nominal_value=1  vc_nominal_unit=V
  C410_100nF : fl_lib/Electrical/Electrical Elements/Capacitor  c=100e-9 F  r=1e-6 Ohm  g=0 1/Ohm  i_specify=off  i_priority=None  i=0 A  i_nominal_specify=off  i_nominal_value=1  i_nominal_unit=A  v_specify=off  v_priority=None  v=0 V  v_nominal_specify=off  v_nominal_value=1  v_nominal_unit=V  vc_specify=off  vc_priority=High  vc=0 V  vc_nominal_specify=off  vc_nominal_value=1  vc_nominal_unit=V
  Electrical Reference{1..4} (4 alike) : fl_lib/Electrical/Electrical Elements/Electrical Reference
  PS-Simulink Converter{,1..4} (5 alike) : nesl_utility/PS-Simulink Converter  PhysicalDomain=network_engine_domain  SubClassName=ps_output  LeftPortType=input  RightPortType=output  PseudoPeriodic=off  Frequencies=[]  VectorFormat=1-D array  Unit=V  AffineConversion=off
  R417-1k : fl_lib/Electrical/Electrical Elements/Resistor  R=1e3 Ohm  i_specify=off  i_priority=None  i=0 A  i_nominal_specify=off  i_nominal_value=1  i_nominal_unit=A  v_specify=off  v_priority=None  v=0 V  v_nominal_specify=off  v_nominal_value=1  v_nominal_unit=V
  R418-12k : fl_lib/Electrical/Electrical Elements/Resistor  R=12e3 Ohm  i_specify=off  i_priority=None  i=0 A  i_nominal_specify=off  i_nominal_value=1  i_nominal_unit=A  v_specify=off  v_priority=None  v=0 V  v_nominal_specify=off  v_nominal_value=1  v_nominal_unit=V
  R421-10k : fl_lib/Electrical/Electrical Elements/Resistor  R=10e3 Ohm  i_specify=off  i_priority=None  i=0 A  i_nominal_specify=off  i_nominal_value=1  i_nominal_unit=A  v_specify=off  v_priority=None  v=0 V  v_nominal_specify=off  v_nominal_value=1  v_nominal_unit=V
  R424-1k : fl_lib/Electrical/Electrical Elements/Resistor  R=1e3 Ohm  i_specify=off  i_priority=None  i=0 A  i_nominal_specify=off  i_nominal_value=1  i_nominal_unit=A  v_specify=off  v_priority=None  v=0 V  v_nominal_specify=off  v_nominal_value=1  v_nominal_unit=V
  R425-12k : fl_lib/Electrical/Electrical Elements/Resistor  R=12e3 Ohm  i_specify=off  i_priority=None  i=0 A  i_nominal_specify=off  i_nominal_value=1  i_nominal_unit=A  v_specify=off  v_priority=None  v=0 V  v_nominal_specify=off  v_nominal_value=1  v_nominal_unit=V
  R426-10k : fl_lib/Electrical/Electrical Elements/Resistor  R=10e3 Ohm  i_specify=off  i_priority=None  i=0 A  i_nominal_specify=off  i_nominal_value=1  i_nominal_unit=A  v_specify=off  v_priority=None  v=0 V  v_nominal_specify=off  v_nominal_value=1  v_nominal_unit=V
  R429-10R : fl_lib/Electrical/Electrical Elements/Resistor  R=10 Ohm  i_specify=off  i_priority=None  i=0 A  i_nominal_specify=off  i_nominal_value=1  i_nominal_unit=A  v_specify=off  v_priority=None  v=0 V  v_nominal_specify=off  v_nominal_value=1  v_nominal_unit=V
  Voltage Sensor{,1..4} (5 alike) : fl_lib/Electrical/Electrical Sensors/Voltage Sensor
  blider_100R : fl_lib/Electrical/Electrical Elements/Resistor  R=100 Ohm  i_specify=off  i_priority=None  i=0 A  i_nominal_specify=off  i_nominal_value=1  i_nominal_unit=A  v_specify=off  v_priority=None  v=0 V  v_nominal_specify=off  v_nominal_value=1  v_nominal_unit=V
  opa-2350 : Subsystem  mask{V_opamp_pos=3.6, V_opamp_neg=-1.6, A=open_loop_gain_opa350}
      mask prompts: V_opamp_pos "V+"; V_opamp_neg "V-"; A "Open Loop Gain"
      mask help: rail to rail op-amp
      mask Help: eval('open opa2350.pdf')
      mask Display:
      | disp('OPA-2350');
      | port_label('lconn', 1, 'in(+)');
      | port_label('lconn', 2, 'in(-)');
      | port_label('rconn', 1, 'out');
  u12 : Scope  NumInputPorts=2
  u23 : Scope  NumInputPorts=2
  uout_circuit_2 : Scope
  u+ : PMIOPort  Side=Left
  u- : PMIOPort  Port=2  Side=Left
  tag scope: u_out_mb_with_howland=global
  wires:
  PS-Simulink Converter3/1 -> u23/1
  PS-Simulink Converter4/1 -> u23/2
  PS-Simulink Converter2/1 -> u12/2
  PS-Simulink Converter1/1 -> u12/1
  PS-Simulink Converter/1 -> [u_out_mb_with_howland], uout_circuit_2/1
  connections:
  Voltage Sensor3/RConn1 -- PS-Simulink Converter3/LConn1
  Voltage Sensor4/RConn1 -- PS-Simulink Converter4/LConn1
  Voltage Sensor4/RConn2 -- Electrical Reference4/LConn1 -- Voltage Sensor3/RConn2
  Voltage Sensor2/RConn1 -- PS-Simulink Converter2/LConn1
  Electrical Reference3/LConn1 -- Voltage Sensor2/RConn2 -- Voltage Sensor1/RConn2
  Voltage Sensor1/RConn1 -- PS-Simulink Converter1/LConn1
  PS-Simulink Converter/LConn1 -- Voltage Sensor/RConn1
  Voltage Sensor/RConn2 -- Electrical Reference1/LConn1
  Voltage Sensor/LConn1 -- R426-10k/RConn1 -- C410_100nF/RConn1 -- R429-10R/RConn1
  R421-10k/RConn1 -- C407_100nF/RConn1 -- Electrical Reference2/LConn1
  R418-12k/LConn1 -- R421-10k/LConn1 -- C407_100nF/LConn1 -- Voltage Sensor4/LConn1 -- opa-2350/LConn1
  R425-12k/RConn1 -- R424-1k/LConn1 -- Voltage Sensor2/LConn1
  R418-12k/RConn1 -- R417-1k/LConn1 -- Voltage Sensor1/LConn1
  C408_100nF/RConn1 -- R424-1k/RConn1 -- blider_100R/RConn1 -- u-/RConn1
  C408_100nF/LConn1 -- R417-1k/RConn1 -- blider_100R/LConn1 -- u+/RConn1
  R426-10k/LConn1 -- Voltage Sensor3/LConn1 -- R425-12k/LConn1 -- C410_100nF/LConn1 -- opa-2350/LConn2
  R429-10R/LConn1 -- opa-2350/RConn1
